simulink model "GaN_Behavioral_Electrothermal_Snapshot"  (R2022b)
settings: Solver=ode45  StartTime=0.0  StopTime=55e-6  MaxStep=5e-9  RelTol=1e-7  AbsTol=1e-8
model workspace (MAT data in the model file):
  C = [8e-05 0.00074 0.0065 0.002]
  R = [0.015 0.23 0.24 0.015]
  p.VDC = 150
  p.L = 9e-05
  p.Cdc = 0.0005
  p.Ron = 0.08
  p.Rdut = 0.0735628553409
  p.Raux = 0.08
  p.Rshunt = 0.01
  p.Rload = 0.001
  p.T0 = 2e-06
  p.Tcharge = 1.8e-05
  p.Tfree = 1e-06
  p.Tmeasure = 5e-06
  p.direction = 1
  p.conventional = 0
  p.idleUpper = 1
values from neighbouring files (symbols this model uses):
  p = evalin(w,'p')    [run_integrated_snapshots.m]
libraries: spsIdealSwitchLib x5, spsSeriesRLCBranchLib x3, spsVoltageMeasurementLib x2, spsCurrentMeasurementLib x2, spsGroundLib x1, spspowerguiLib x1
settings Model: Creator=Greatlovers  LastModifiedBy=Greatlovers

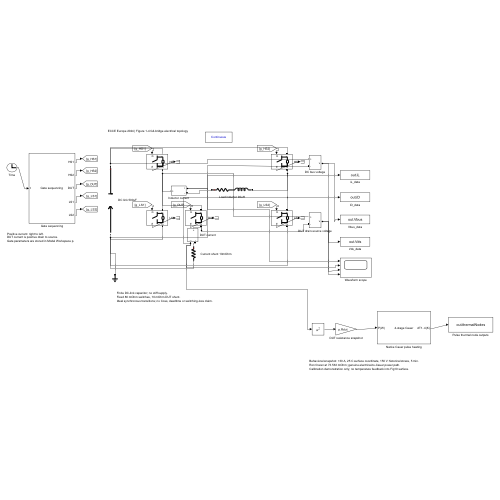
[thumbnail: Simulink's stored preview of the top-level diagram]
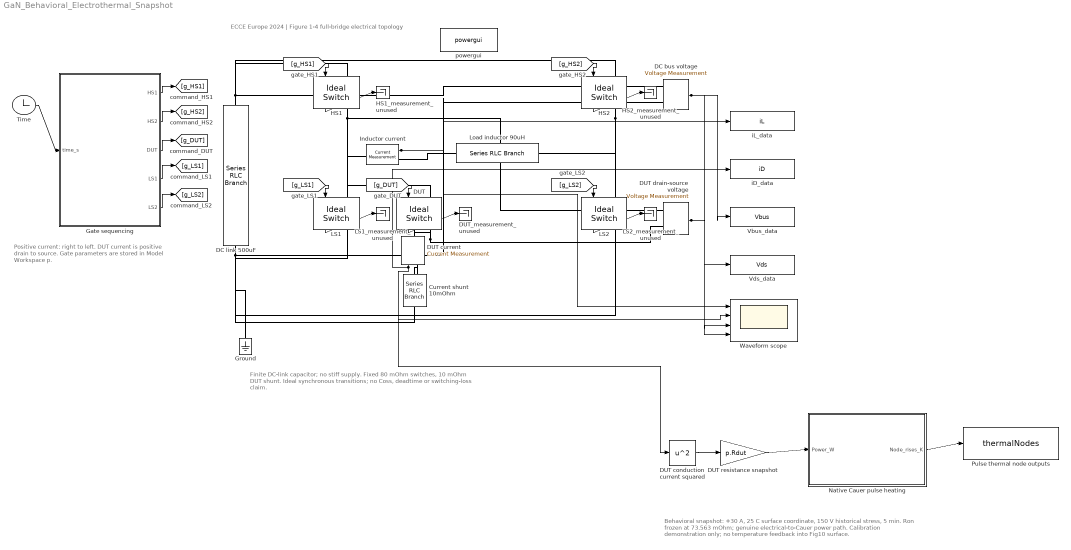
== system GaN_Behavioral_Electrothermal_Snapshot ==
  note: ECCE Europe 2024 | Figure 1-4 full-bridge electrical topology
  note: Finite DC-link capacitor; no stiff supply.
      | Fixed 80 mOhm switches, 10 mOhm DUT shunt.
      | Ideal synchronous transitions; no Coss, deadtime or switching-loss claim.
  note: Positive current: right to left.
      | DUT current is positive drain to source.
      | Gate parameters are stored in Model Workspace p.
  note: Behavioral snapshot: +30 A, 25 C surface coordinate, 150 V historical stress, 5 min.
      | Ron frozen at 73.563 mOhm; genuine electrical-to-Cauer power path.
      | Calibration demonstration only; no temperature feedback into Fig10 surface.
  Current shunt 10mOhm : spsSeriesRLCBranchLib/Series RLC Branch  LConnTagsString=__new0  RConnTagsString=__new0  BranchType=R  Resistance=p.Rshunt  Inductance=1e-3  SetiL0=off  InitialCurrent=0  Capacitance=1e-6  Setx0=off  InitialVoltage=0  Measurements=None
  DC bus voltage : spsVoltageMeasurementLib/Voltage Measurement  PhasorSimulation=off  OutputType=Complex  PSBequivalent=0
  DC link 500uF : spsSeriesRLCBranchLib/Series RLC Branch  LConnTagsString=__new0  RConnTagsString=__new0  BranchType=C  Resistance=1  Inductance=1e-3  SetiL0=off  InitialCurrent=0  Capacitance=p.Cdc  Setx0=on  InitialVoltage=p.VDC  Measurements=None
  DUT : spsIdealSwitchLib/Ideal Switch  Ron=p.Rdut  Lon=0  IC=0  Rs=1e9  Cs=inf  Measurements=on
  DUT conduction current squared : Math  Operator=square
  DUT current : spsCurrentMeasurementLib/Current Measurement  PhasorSimulation=off  OutputType=Complex  PSBequivalent=0
  DUT drain-source voltage : spsVoltageMeasurementLib/Voltage Measurement  PhasorSimulation=off  OutputType=Complex  PSBequivalent=0
  DUT resistance snapshot : Gain  Gain=p.Rdut
  DUT_measurement_unused : Terminator
  Gate sequencing : Subsystem
      mask Display: disp('Gate sequencing');port_label('input',1,'t');port_label('output',1,'HS1');port_label('output',2,'HS2');port_label('output',3,'DUT');port_label('output',4,'LS1');port_label('output',5,'LS2');
  Ground : spsGroundLib/Ground  LConnTagsString=a
  HS1 : spsIdealSwitchLib/Ideal Switch  Ron=p.Raux  Lon=0  IC=0  Rs=1e9  Cs=inf  Measurements=on
  HS1_measurement_unused : Terminator
  HS2 : spsIdealSwitchLib/Ideal Switch  Ron=p.Raux  Lon=0  IC=0  Rs=1e9  Cs=inf  Measurements=on
  HS2_measurement_unused : Terminator
  Inductor current : spsCurrentMeasurementLib/Current Measurement  PhasorSimulation=off  OutputType=Complex  PSBequivalent=0
  LS1 : spsIdealSwitchLib/Ideal Switch  Ron=p.Raux  Lon=0  IC=0  Rs=1e9  Cs=inf  Measurements=on
  LS1_measurement_unused : Terminator
  LS2 : spsIdealSwitchLib/Ideal Switch  Ron=p.Raux  Lon=0  IC=0  Rs=1e9  Cs=inf  Measurements=on
  LS2_measurement_unused : Terminator
  Load inductor 90uH : spsSeriesRLCBranchLib/Series RLC Branch  LConnTagsString=__new0  RConnTagsString=__new0  BranchType=RL  Resistance=p.Rload  Inductance=p.L  SetiL0=on  InitialCurrent=0  Capacitance=1e-6  Setx0=off  InitialVoltage=0  Measurements=None
  Native Cauer pulse heating : Subsystem
      mask Display: disp('4-stage Cauer');port_label('input',1,'P(W)');port_label('output',1,'dT1..4(K)');
  Pulse thermal node outputs : ToWorkspace  VariableName=thermalNodes  SaveFormat=Timeseries  SampleTime=-1
  Time : Clock
  Vbus_data : ToWorkspace  VariableName=Vbus  SaveFormat=Timeseries  SampleTime=-1
  Vds_data : ToWorkspace  VariableName=Vds  SaveFormat=Timeseries  SampleTime=-1
  Waveform scope : Scope  NumInputPorts=4
  iD_data : ToWorkspace  VariableName=iD  SaveFormat=Timeseries  SampleTime=-1
  iL_data : ToWorkspace  VariableName=iL  SaveFormat=Timeseries  SampleTime=-1
  powergui : spspowerguiLib/powergui  Priority=1  SimulationMode=Continuous  SampleTime=50e-6  frequency=60  Iterations=50  frequencyindice=60  Pbase=100e6  ErrMax=1e-4  UnitsV=kV  UnitsW=MW  buscounter=0  FunctionMessages=off  echomessages=off  EnableUseOfTLC=off  CurrentSourceSwitches=off  DisableSnubberDevices=off  DisableRonSwitches=off  DisableVfSwitches=off  DisplayEquations=off  AutomaticDiscreteSolvers=off  SolverType=Tustin/Backward Euler (TBE)  Interpol=off  ExternalGateDelay=off  methode=off  Ts=100  x0status=blocks  SPID=on  SwTol=0  HookPort=off  NonlinearTolerance=1e-4  nMaxIteration=100  ContinueOnMaxIteration=off  RestoreLinks=warning  ResistiveCurrentMeasurement=off  Frange=[0:2:500]  Ylog=off  Xlog=on  ShowGrid=off  save=off  variable=ZData  structure=0  ZoomFFT=off  StartTime=0.0  cycles=1  DisplayStyle=1  fundamental=60  FreqAxis=off  MaxFrequency=1000  frequencyindicesteady=1  RmsSteady=1  display=off
  wires:
  Time/1 -> Gate sequencing/1(time_s)
  HS1/1 -> HS1_measurement_unused/1
  HS2/1 -> HS2_measurement_unused/1
  DUT/1 -> DUT_measurement_unused/1
  LS1/1 -> LS1_measurement_unused/1
  LS2/1 -> LS2_measurement_unused/1
  Inductor current/1 -> iL_data/1, Waveform scope/1
  DUT current/1 -> iD_data/1, Waveform scope/2, DUT conduction current squared/1
  DC bus voltage/1 -> Vbus_data/1, Waveform scope/3
  DUT drain-source voltage/1 -> Vds_data/1, Waveform scope/4
  Gate sequencing/1(HS1) -> [g_HS1]
  [g_HS1] -> HS1/1
  Gate sequencing/2(HS2) -> [g_HS2]
  [g_HS2] -> HS2/1
  Gate sequencing/3(DUT) -> [g_DUT]
  [g_DUT] -> DUT/1
  Gate sequencing/4(LS1) -> [g_LS1]
  [g_LS1] -> LS1/1
  Gate sequencing/5(LS2) -> [g_LS2]
  [g_LS2] -> LS2/1
  DUT conduction current squared/1 -> DUT resistance snapshot/1
  DUT resistance snapshot/1 -> Native Cauer pulse heating/1(Power_W)
  Native Cauer pulse heating/1(Node_rises_K) -> Pulse thermal node outputs/1
  connections:
  HS1/LConn1 -- DC link 500uF/LConn1 -- HS2/LConn1 -- DC bus voltage/LConn1
  LS1/LConn1 -- HS1/RConn1 -- DUT/LConn1 -- Inductor current/LConn1 -- DUT drain-source voltage/LConn1
  Inductor current/RConn1 -- Load inductor 90uH/LConn1
  HS2/RConn1 -- Load inductor 90uH/RConn1 -- LS2/LConn1
  DUT current/LConn1 -- DUT/RConn1 -- DUT drain-source voltage/LConn2
  DUT current/RConn1 -- Current shunt 10mOhm/LConn1
  LS1/RConn1 -- DC link 500uF/RConn1 -- LS2/RConn1 -- Current shunt 10mOhm/RConn1 -- Ground/LConn1 -- DC bus voltage/LConn2

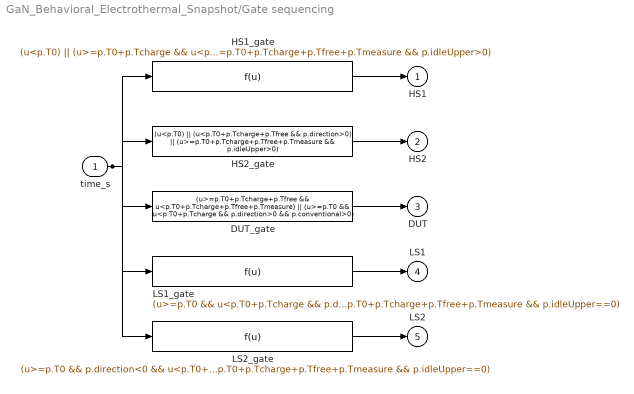
== system GaN_Behavioral_Electrothermal_Snapshot/Gate sequencing ==
  time_s : Inport
  DUT_gate : Fcn  Expr=(u>=p.T0+p.Tcharge+p.Tfree && u<p.T0+p.Tcharge+p.Tfree+p.Tmeasure) || (u>=p.T0 && u<p.T0+p.Tcharge && p.direction>0 && p.conventional>0)
  HS1_gate : Fcn  Expr=(u<p.T0) || (u>=p.T0+p.Tcharge && u<p.T0+p.Tcharge+p.Tfree && p.direction>0) || (u>=p.T0 && u<p.T0+p.Tcharge && p.direction<0) || (u>=p.T0+p.Tcharge+p.Tfree+p.Tmeasure && p.idleUpper>0)
  HS2_gate : Fcn  Expr=(u<p.T0) || (u<p.T0+p.Tcharge+p.Tfree && p.direction>0) || (u>=p.T0+p.Tcharge+p.Tfree+p.Tmeasure && p.idleUpper>0)
  LS1_gate : Fcn  Expr=(u>=p.T0 && u<p.T0+p.Tcharge && p.direction>0 && p.conventional==0) || (u>=p.T0+p.Tcharge+p.Tfree+p.Tmeasure && p.idleUpper==0)
  LS2_gate : Fcn  Expr=(u>=p.T0 && p.direction<0 && u<p.T0+p.Tcharge+p.Tfree+p.Tmeasure) || (u>=p.T0+p.Tcharge+p.Tfree && u<p.T0+p.Tcharge+p.Tfree+p.Tmeasure) || (u>=p.T0+p.Tcharge+p.Tfree+p.Tmeasure && p.idleUpper==0)
  HS1 : Outport
  HS2 : Outport  Port=2
  DUT : Outport  Port=3
  LS1 : Outport  Port=4
  LS2 : Outport  Port=5
  wires:
  time_s/1 -> HS1_gate/1, HS2_gate/1, DUT_gate/1, LS1_gate/1, LS2_gate/1
  HS1_gate/1 -> HS1/1
  HS2_gate/1 -> HS2/1
  DUT_gate/1 -> DUT/1
  LS1_gate/1 -> LS1/1
  LS2_gate/1 -> LS2/1

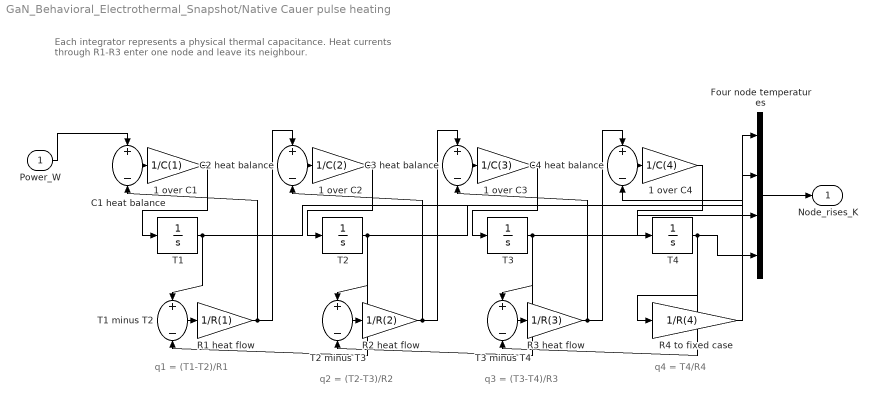
== system GaN_Behavioral_Electrothermal_Snapshot/Native Cauer pulse heating ==
  note: q4 = T4/R4
  note: q3 = (T3-T4)/R3
  note: q2 = (T2-T3)/R2
  note: q1 = (T1-T2)/R1
  note: Each integrator represents a physical thermal capacitance.
      | Heat currents through R1-R3 enter one node and leave its neighbour.
  Power_W : Inport
  1 over C1 : Gain  Gain=1/C(1)
  1 over C2 : Gain  Gain=1/C(2)
  1 over C3 : Gain  Gain=1/C(3)
  1 over C4 : Gain  Gain=1/C(4)
  C1 heat balance : Sum  Inputs=+-
  C2 heat balance : Sum  Inputs=+-
  C3 heat balance : Sum  Inputs=+-
  C4 heat balance : Sum  Inputs=+-
  Four node temperatures : Mux
  R1 heat flow : Gain  Gain=1/R(1)
  R2 heat flow : Gain  Gain=1/R(2)
  R3 heat flow : Gain  Gain=1/R(3)
  R4 to fixed case : Gain  Gain=1/R(4)
  T{1..4} (4 alike) : Integrator
  T1 minus T2 : Sum  Inputs=+-
  T2 minus T3 : Sum  Inputs=+-
  T3 minus T4 : Sum  Inputs=+-
  Node_rises_K : Outport
  wires:
  Four node temperatures/1 -> Node_rises_K/1
  R4 to fixed case/1 -> C4 heat balance/2
  R3 heat flow/1 -> C4 heat balance/1, C3 heat balance/2
  T3 minus T4/1 -> R3 heat flow/1
  T4/1 -> Four node temperatures/4, R4 to fixed case/1, T3 minus T4/2
  R2 heat flow/1 -> C3 heat balance/1, C2 heat balance/2
  T2 minus T3/1 -> R2 heat flow/1
  T3/1 -> Four node temperatures/3, T3 minus T4/1, T2 minus T3/2
  R1 heat flow/1 -> C2 heat balance/1, C1 heat balance/2
  T1 minus T2/1 -> R1 heat flow/1
  T2/1 -> Four node temperatures/2, T2 minus T3/1, T1 minus T2/2
  T1/1 -> Four node temperatures/1, T1 minus T2/1
  Power_W/1 -> C1 heat balance/1
  1 over C4/1 -> T4/1
  C4 heat balance/1 -> 1 over C4/1
  1 over C3/1 -> T3/1
  C3 heat balance/1 -> 1 over C3/1
  1 over C2/1 -> T2/1
  C2 heat balance/1 -> 1 over C2/1
  1 over C1/1 -> T1/1
  C1 heat balance/1 -> 1 over C1/1
